simulink model "mamba_f405_quadcopter"  (R2024b)
settings: Solver=ode1  StartTime=0.0  StopTime=6.0  FixedStep=0.001  RelTol=1e-3
settings Model: Creator=djall  LastModifiedBy=djall

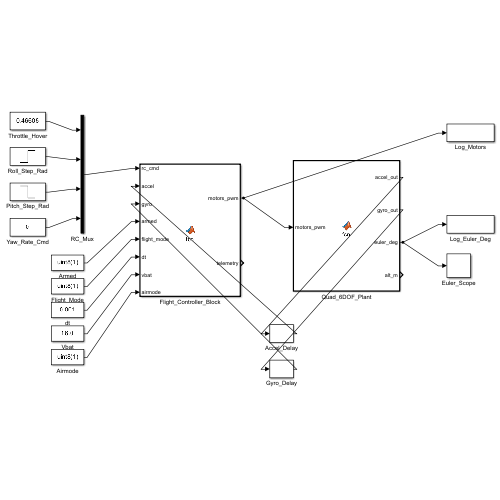
[thumbnail: Simulink's stored preview of the top-level diagram]
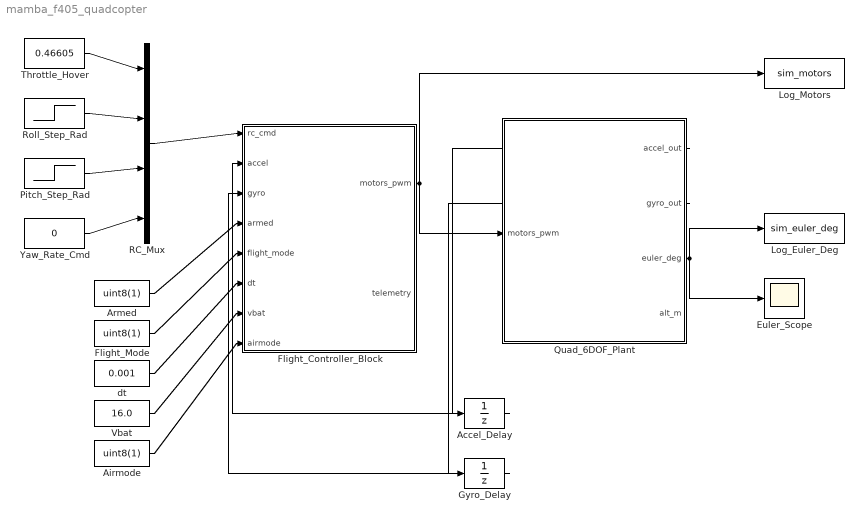
== system mamba_f405_quadcopter ==
  Accel_Delay : UnitDelay  InitialCondition=[0; 0; 9.81]  SampleTime=0.001  HasFrameUpgradeWarning=on
  Airmode : Constant  Value=uint8(1)
  Armed : Constant  Value=uint8(1)
  Euler_Scope : Scope
  Flight_Controller_Block : MATLAB Function  TreatAsAtomicUnit=on
  Flight_Mode : Constant  Value=uint8(1)
  Gyro_Delay : UnitDelay  InitialCondition=[0; 0; 0]  SampleTime=0.001  HasFrameUpgradeWarning=on
  Log_Euler_Deg : ToWorkspace  VariableName=sim_euler_deg  SaveFormat=Timeseries  SampleTime=-1
  Log_Motors : ToWorkspace  VariableName=sim_motors  SaveFormat=Timeseries  SampleTime=-1
  Pitch_Step_Rad : Step  Time=3.5  After=-0.2618  SampleTime=0.001
  Quad_6DOF_Plant : MATLAB Function  TreatAsAtomicUnit=on
  RC_Mux : Mux
  Roll_Step_Rad : Step  Time=1.5  After=0.2618  SampleTime=0.001
  Throttle_Hover : Constant  Value=0.46605
  Vbat : Constant  Value=16.0
  Yaw_Rate_Cmd : Constant  Value=0
  dt : Constant  Value=0.001
  wires:
  Throttle_Hover/1 -> RC_Mux/1
  Roll_Step_Rad/1 -> RC_Mux/2
  Pitch_Step_Rad/1 -> RC_Mux/3
  Yaw_Rate_Cmd/1 -> RC_Mux/4
  RC_Mux/1 -> Flight_Controller_Block/1(rc_cmd)
  Accel_Delay/1 -> Flight_Controller_Block/2(accel)
  Gyro_Delay/1 -> Flight_Controller_Block/3(gyro)
  Armed/1 -> Flight_Controller_Block/4(armed)
  Flight_Mode/1 -> Flight_Controller_Block/5(flight_mode)
  dt/1 -> Flight_Controller_Block/6(dt)
  Vbat/1 -> Flight_Controller_Block/7(vbat)
  Airmode/1 -> Flight_Controller_Block/8(airmode)
  Flight_Controller_Block/1(motors_pwm) -> Quad_6DOF_Plant/1(motors_pwm), Log_Motors/1
  Quad_6DOF_Plant/1(accel_out) -> Accel_Delay/1
  Quad_6DOF_Plant/2(gyro_out) -> Gyro_Delay/1
  Quad_6DOF_Plant/3(euler_deg) -> Log_Euler_Deg/1, Euler_Scope/1

== matlab function mamba_f405_quadcopter/Quad_6DOF_Plant ==
  data: motors_pwm input; accel_out output; gyro_out output; euler_deg output; alt_m output
function [accel_out, gyro_out, euler_deg, alt_m] = plant(motors_pwm)
persistent pos vel q omega rotor_omega;
if isempty(pos)
    pos = [0;0;0]; vel = [0;0;0]; q = [1;0;0;0]; omega = [0;0;0];
    rotor_omega = [200;200;200;200];
end
dt = 0.001; m = 0.650; g = 9.81; d = 0.125/sqrt(2);
J = diag([4.85e-3, 4.85e-3, 8.80e-3]); kt = 1.15e-6; km = 1.90e-8;
pwm_norm = max(min((motors_pwm - 1000.0) / 1000.0, 1.0), 0.0);
w_cmd = 200.0 + pwm_norm * 2000.0;
rotor_omega = rotor_omega + (dt / 0.020) * (w_cmd - rotor_omega);
T = kt * (rotor_omega.^2); Q = km * (rotor_omega.^2);
tau = [d*(-T(1)-T(2)+T(3)+T(4)); d*(-T(1)+T(2)-T(3)+T(4)); -Q(1)+Q(2)+Q(3)-Q(4)] - 0.0025*omega;
omega = omega + (J \ (tau - cross(omega, J*omega))) * dt;
q0=q(1); q1=q(2); q2=q(3); q3=q(4); p=omega(1); qr=omega(2); r=omega(3);
q = q + 0.5*[-q1*p-q2*qr-q3*r; q0*p+q2*r-q3*qr; q0*qr-q1*r+q3*p; q0*r+q1*qr-q2*p]*dt;
q = q / norm(q);
q0=q(1); q1=q(2); q2=q(3); q3=q(4);
R_IB = [1-2*(q2^2+q3^2), 2*(q1*q2-q0*q3), 2*(q1*q3+q0*q2);
        2*(q1*q2+q0*q3), 1-2*(q1^2+q3^2), 2*(q2*q3-q0*q1);
        2*(q1*q3-q0*q2), 2*(q2*q3+q0*q1), 1-2*(q1^2+q2^2)];
acc = (R_IB*[0;0;-sum(T)] + [0;0;m*g] - 0.18*vel) / m;
if pos(3)>=0 && acc(3)>0 && sum(T)<m*g, vel(3)=0; acc(3)=0; pos(3)=0; end
vel = vel + acc*dt; pos = pos + vel*dt;
if pos(3)>0, pos(3)=0; vel(3)=0; end
accel_out = R_IB' * [0;0;g];
gyro_out  = omega;
roll  = atan2(2*(q0*q1+q2*q3), 1-2*(q1^2+q2^2));
pitch = asin(max(min(2*(q0*q2-q3*q1),1),-1));
yaw   = atan2(2*(q0*q3+q1*q2), 1-2*(q2^2+q3^2));
euler_deg = [roll; pitch; yaw] * (180/pi);
alt_m = -pos(3);

== matlab function mamba_f405_quadcopter/Flight_Controller_Block ==
  data: rc_cmd input; motors_pwm output; accel input; gyro input; armed input; flight_mode input; dt input; vbat input; airmode input; telemetry output
function [motors_pwm, telemetry] = fcn(rc_cmd, accel, gyro, armed, flight_mode, dt, vbat, airmode)
coder.extrinsic('flight_controller');
motors_pwm = zeros(4,1);
telemetry = zeros(6,1);
[motors_pwm, telemetry] = flight_controller(rc_cmd, accel, gyro, armed, flight_mode, dt, vbat, airmode);
